simulink model "synRelSimuLutObs"  (R2023b)
settings: Solver=ode4  StartTime=0.0  StopTime=scenario.stopTime  FixedStep=Ts  RelTol=1e-4
values from neighbouring files (symbols this model uses):
  motor = setMotorParameters("SynRelLaplace")    [initSimulinkObs.m]    (also in setMotorParameters.m = struct)
  scenario = struct    [initSimulinkObs.m]
  trajectory = lutData.trajectory    [initSimulinkObs.m]    (also in test_cartos.m = load('synRelSimuLutData.mat').trajectory)
  Ts = 1e-4    (= 0.0001)    [initSimulinkObs.m]
undefined symbols (not defined in the file or in its folder): control, DiscIntNeverNeededParam, inverter, math, observer
libraries: simulink x2, slpidlib x1
settings Model: Creator=promu  LastModifiedBy=peralezADM
settings OptimizationCC: ReuseModelBlockBuffer=off
settings ModelReferenceCC: EnableRefExpFcnMdlSchedulingChecks=on

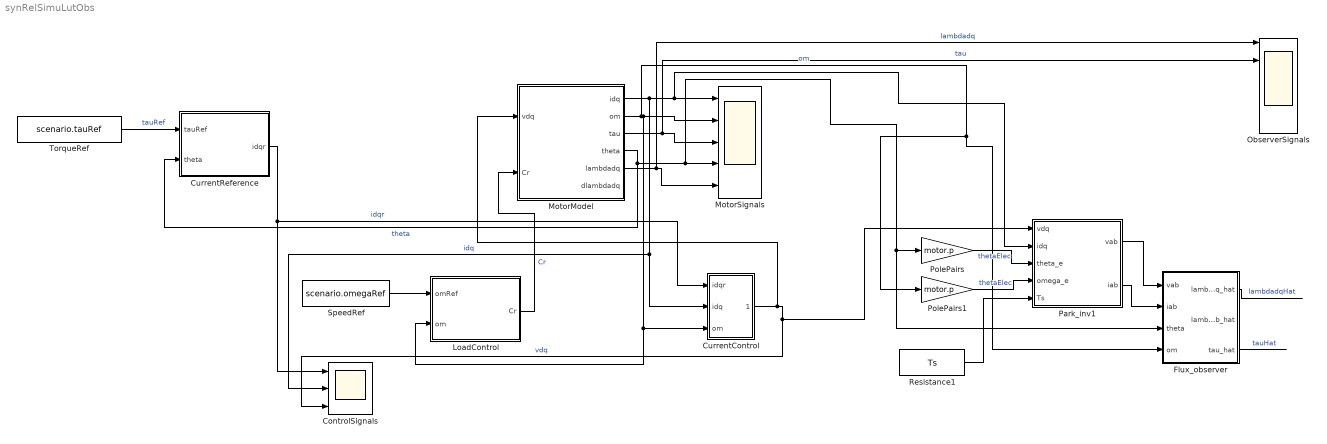
== system synRelSimuLutObs ==
  ControlSignals : Scope  NumInputPorts=3
  CurrentControl : Subsystem
  CurrentReference : Subsystem
  Flux_observer : Subsystem
  LoadControl : Subsystem
  MotorModel : Subsystem
  MotorSignals : Scope  NumInputPorts=5
  ObserverSignals : Scope  NumInputPorts=11
  Park_inv1 : MATLAB Function  TreatAsAtomicUnit=on
  PolePairs : Gain  Gain=motor.p
  PolePairs1 : Gain  Gain=motor.p
  Resistance1 : Constant  Value=Ts
  SpeedRef : Constant  Value=scenario.omegaRef
  TorqueRef : Constant  Value=scenario.tauRef
  wires:
  TorqueRef/1 -> CurrentReference/1(tauRef)  "tauRef"
  LoadControl/1(Cr) -> MotorModel/2(Cr)  "Cr"
  CurrentReference/1(idqr) -> CurrentControl/1(idqr), ControlSignals/1  "idqr"
  CurrentControl/1(v_dq) -> Park_inv1/1(vdq), ControlSignals/3, MotorModel/1(vdq)  "vdq"
  MotorModel/4(theta) -> CurrentReference/2(theta), MotorSignals/4, Flux_observer/3(theta), PolePairs/1  "theta"
  MotorModel/5(lambdadq) -> MotorSignals/5, ObserverSignals/1  "lambdadq"
  MotorModel/3(tau) -> ObserverSignals/3, MotorSignals/3  "tau"
  MotorModel/2(om) -> LoadControl/2(om), CurrentControl/3(om), MotorSignals/2, PolePairs1/1, Flux_observer/4(om)  "om"
  MotorModel/1(idq) -> ControlSignals/2, CurrentControl/2(idq), MotorSignals/1, Park_inv1/2(idq)  "idq"
  SpeedRef/1 -> LoadControl/1(omRef)
  Park_inv1/1(vab) -> Flux_observer/1(vab)
  PolePairs/1 -> Park_inv1/3(theta_e)  "thetaElec"
  Flux_observer/1(lambda_dq_hat) -> ?  "lambdadqHat"
  PolePairs1/1 -> Park_inv1/4(omega_e)  "thetaElec"
  Resistance1/1 -> Park_inv1/5(Ts)
  Park_inv1/2(iab) -> Flux_observer/2(iab)
  Flux_observer/3(tau_hat) -> ?  "tauHat"

== system synRelSimuLutObs/CurrentControl ==
  idqr : Inport
  idq : Inport  Port=2
  om : Inport  Port=3
  FeedbackLinearization : Subsystem
  GainElec : Constant  Value=control.kElecd  OutDataTypeStr=double
  PiCurrentLoops : Subsystem
      settings: PortSchema="{\"entries\":[{\"content\":{\"sides\":[{\"content\":{\"connectorIds\":[\"In1\",\"In2\",\"In3\"]},\"type\":\"ConnectorPlacement.EquallySpacedRectSide\",\"uuid\":\"0dd1bd5c-4f2d-4a51-9bc2-8bf74640d4ff\"},{\"content\":{\"connectorIds\":[\"Out1\"],\"side\":\"RIGHT\"},\"type\":\"ConnectorPlacement.EquallySpacedRectSide\",\"uuid\":\"9ff54608-efe8-47a2-97c0-1c2807ae0451\"},{\"content\":{\"connectorIds\":[],\"side\":\"TOP\"},\"type\":\"ConnectorPlacement.EquallySpacedRectSide\",\"uuid\":\"a5b0a1bc-2629-443b-a6ad-4c332df72e2c\"},{\"content\":{\"connectorIds\":[\"In4\",\"In5\"],\"side\":\"BOTTOM\"},\"type\":\"ConnectorPlacement.EquallySpacedRectSide\",\"uuid\":\"e8d63822-9705-4716-821c-9412f2966827\"},{\"content\":{\"connectorIds\":[],\"side\":\"HIDDEN\"},\"type\":\"ConnectorPlacement.EquallySpacedRectSide\",\"uuid\":\"63401b5c-75e9-49e9-aa08-12658d9987d3\"}]},\"type\":\"ConnectorPlacement.EquallySpacedConnector\",\"uuid\":\"d3f45542-3ea7-483a-a2ee-6c72d9ae8820\"}],\"packageUris\":[\"http://schema.mathworks.com/mf0/Connector/R2020b\"],\"version\":\"1.0\"}"
  VoltageSaturation : Subsystem
  v_dq : Outport
  wires:
  VoltageSaturation/1(vdqsat) -> v_dq/1
  FeedbackLinearization/1(v_dq) -> VoltageSaturation/1(vdq)
  idq/1 -> FeedbackLinearization/1(idq), PiCurrentLoops/2(idq)
  PiCurrentLoops/1(v_dq) -> FeedbackLinearization/2(udq)
  idqr/1 -> PiCurrentLoops/1(idqr)
  om/1 -> FeedbackLinearization/3(om)
  GainElec/1 -> PiCurrentLoops/5(Keq), PiCurrentLoops/4(Ked)
  VoltageSaturation/2(saturation) -> PiCurrentLoops/3(saturation)

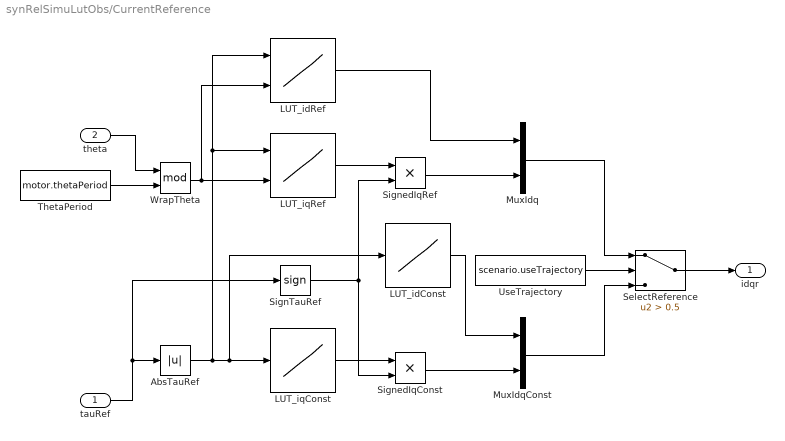
== system synRelSimuLutObs/CurrentReference ==
  tauRef : Inport
  theta : Inport  Port=2
  AbsTauRef : Abs  SaturateOnIntegerOverflow=off
  LUT_idConst : Lookup_n-D  NumberOfTableDimensions=1  BreakpointsForDimension1=trajectory.tauRef  Table=trajectory.idConst  ExtrapMethod=Clip  InternalRulePriority=Speed  RndMeth=Simplest
  LUT_idRef : Lookup_n-D  BreakpointsForDimension1=trajectory.tauRef  BreakpointsForDimension2=trajectory.theta  Table=trajectory.id  ExtrapMethod=Clip  InternalRulePriority=Speed  RndMeth=Simplest
      settings: InputPortMap=u0,u1
  LUT_iqConst : Lookup_n-D  NumberOfTableDimensions=1  BreakpointsForDimension1=trajectory.tauRef  Table=trajectory.iqConst  ExtrapMethod=Clip  InternalRulePriority=Speed  RndMeth=Simplest
  LUT_iqRef : Lookup_n-D  BreakpointsForDimension1=trajectory.tauRef  BreakpointsForDimension2=trajectory.theta  Table=trajectory.iq  ExtrapMethod=Clip  InternalRulePriority=Speed  RndMeth=Simplest
      settings: InputPortMap=u0,u1
  MuxIdq : Mux  Inputs=2
  MuxIdqConst : Mux  Inputs=2
  SelectReference : Switch  Criteria=u2 > Threshold  Threshold=0.5  SaturateOnIntegerOverflow=off  InputSameDT=off
  SignTauRef : Signum
  SignedIqConst : Product
  SignedIqRef : Product
  ThetaPeriod : Constant  Value=motor.thetaPeriod
  UseTrajectory : Constant  Value=scenario.useTrajectory
  WrapTheta : Math  Operator=mod
  idqr : Outport
  wires:
  MuxIdqConst/1 -> SelectReference/3
  UseTrajectory/1 -> SelectReference/2
  theta/1 -> WrapTheta/1
  SelectReference/1 -> idqr/1
  LUT_idConst/1 -> MuxIdqConst/1
  ThetaPeriod/1 -> WrapTheta/2
  tauRef/1 -> AbsTauRef/1, SignTauRef/1
  LUT_idRef/1 -> MuxIdq/1
  SignedIqConst/1 -> MuxIdqConst/2
  WrapTheta/1 -> LUT_iqRef/2, LUT_idRef/2
  AbsTauRef/1 -> LUT_iqConst/1, LUT_idConst/1, LUT_idRef/1, LUT_iqRef/1
  LUT_iqRef/1 -> SignedIqRef/1
  LUT_iqConst/1 -> SignedIqConst/1
  SignedIqRef/1 -> MuxIdq/2
  SignTauRef/1 -> SignedIqRef/2, SignedIqConst/2
  MuxIdq/1 -> SelectReference/1

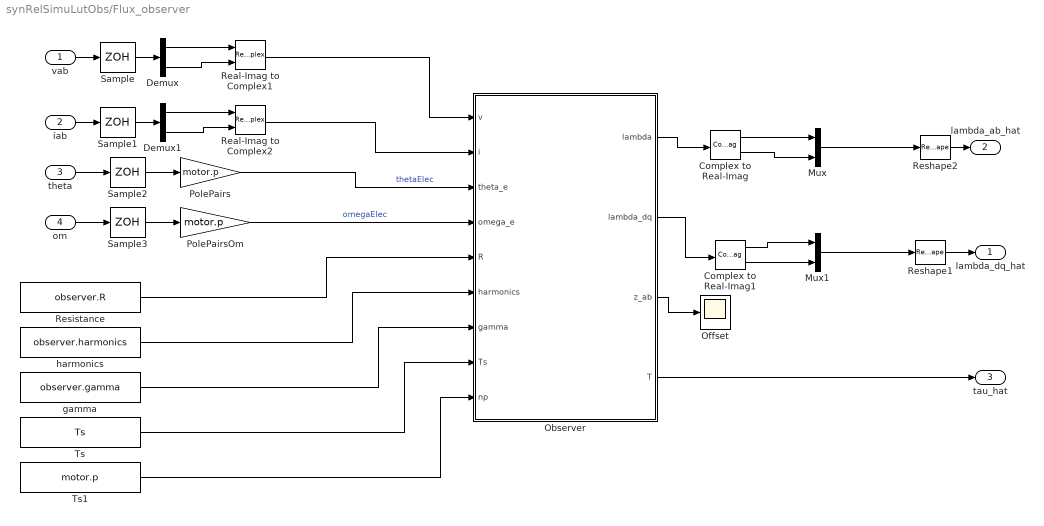
== system synRelSimuLutObs/Flux_observer ==
  vab : Inport
  iab : Inport  Port=2
  theta : Inport  Port=3
  om : Inport  Port=4
  Complex to Real-Imag : ComplexToRealImag
  Complex to Real-Imag1 : ComplexToRealImag
  Demux : Demux  Outputs=2
  Demux1 : Demux  Outputs=2
  Mux : Mux  Inputs=2
  Mux1 : Mux  Inputs=2
  Observer : MATLAB Function  TreatAsAtomicUnit=on
  Offset : Scope
  PolePairs : Gain  Gain=motor.p
  PolePairsOm : Gain  Gain=motor.p
  Real-Imag to Complex1 : RealImagToComplex
  Real-Imag to Complex2 : RealImagToComplex
  Reshape1 : Reshape
  Reshape2 : Reshape
  Resistance : Constant  Value=observer.R
  Sample{,1..3} (4 alike) : ZeroOrderHold  SampleTime=Ts
  Ts : Constant  Value=Ts
  Ts1 : Constant  Value=motor.p
  gamma : Constant  Value=observer.gamma
  harmonics : Constant  Value=observer.harmonics
  lambda_dq_hat : Outport
  lambda_ab_hat : Outport  Port=2
  tau_hat : Outport  Port=3
  wires:
  theta/1 -> Sample2/1
  om/1 -> Sample3/1
  PolePairsOm/1 -> Observer/4(omega_e)  "omegaElec"
  Resistance/1 -> Observer/5(R)
  harmonics/1 -> Observer/6(harmonics)
  gamma/1 -> Observer/7(gamma)
  PolePairs/1 -> Observer/3(theta_e)  "thetaElec"
  Mux1/1 -> Reshape1/1
  Reshape1/1 -> lambda_dq_hat/1
  Reshape2/1 -> lambda_ab_hat/1
  vab/1 -> Sample/1
  Demux/2 -> Real-Imag to Complex1/2
  Demux/1 -> Real-Imag to Complex1/1
  Real-Imag to Complex1/1 -> Observer/1(v)
  iab/1 -> Sample1/1
  Demux1/1 -> Real-Imag to Complex2/1
  Demux1/2 -> Real-Imag to Complex2/2
  Real-Imag to Complex2/1 -> Observer/2(i)
  Observer/1(lambda) -> Complex to Real-Imag/1
  Complex to Real-Imag/2 -> Mux/2
  Complex to Real-Imag/1 -> Mux/1
  Ts/1 -> Observer/8(Ts)
  Mux/1 -> Reshape2/1
  Observer/2(lambda_dq) -> Complex to Real-Imag1/1
  Complex to Real-Imag1/2 -> Mux1/2
  Complex to Real-Imag1/1 -> Mux1/1
  Observer/3(z_ab) -> Offset/1
  Sample/1 -> Demux/1
  Sample1/1 -> Demux1/1
  Sample2/1 -> PolePairs/1
  Sample3/1 -> PolePairsOm/1
  Ts1/1 -> Observer/9(np)
  Observer/4(T) -> tau_hat/1

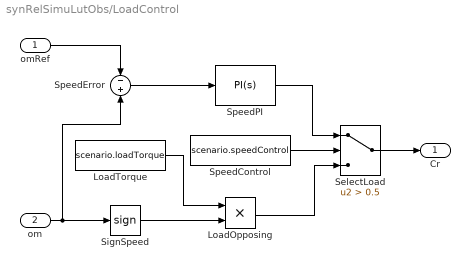
== system synRelSimuLutObs/LoadControl ==
  omRef : Inport
  om : Inport  Port=2
  LoadOpposing : Product
  LoadTorque : Constant  Value=scenario.loadTorque
  SelectLoad : Switch  Criteria=u2 > Threshold  Threshold=0.5  SaturateOnIntegerOverflow=off  InputSameDT=off
  SignSpeed : Signum
  SpeedControl : Constant  Value=scenario.speedControl
  SpeedError : Sum  Inputs=-+
  SpeedPI : slpidlib/PID Controller  Controller=PI  Form=Parallel  TimeDomain=Continuous-time  UseExternalTs=off  SampleTime=-1  IntegratorMethod=Forward Euler  FilterMethod=Forward Euler  ControllerParametersSource=internal  P=control.kpSpeed  I=control.kiSpeed  UseKiTs=off  D=0  N=100  UseFilter=on  TunerSelectOption=Transfer Function Based (PID Tuner App)  InitialConditionSource=internal  InitialConditionForIntegrator=0  InitialConditionForFilter=0  DifferentiatorICPrevScaledInput=0  ExternalReset=none  TrackingMode=off  Kt=1  LimitOutput=on  SatLimitsSource=internal  UpperSaturationLimit=scenario.loadMax  LowerSaturationLimit=-scenario.loadMax  LinearizeAsGain=on  AntiWindupMode=clamping  Kb=1  LimitIntegrator=off  UpperIntegratorSaturationLimit=inf  LowerIntegratorSaturationLimit=-inf  POutMin=[]  POutMax=[]  IOutMin=[]  IOutMax=[]  DOutMin=[]  DOutMax=[]  NOutMin=[]  NOutMax=[]  SumOutMin=[]  SumOutMax=[]  SaturationOutMin=[]  SaturationOutMax=[]  PParamMin=[]  PParamMax=[]  IParamMin=[]  IParamMax=[]  DParamMin=[]  DParamMax=[]  NParamMin=[]  NParamMax=[]  KbParamMin=[]  KbParamMax=[]  KtParamMin=[]  KtParamMax=[]  KbOutMin=[]  KbOutMax=[]  KtOutMin=[]  KtOutMax=[]  IntegratorOutMin=[]  IntegratorOutMax=[]  FilterOutMin=[]  FilterOutMax=[]  SumI1OutMin=[]  SumI1OutMax=[]  SumI2OutMin=[]  SumI2OutMax=[]  SumI3OutMin=[]  SumI3OutMax=[]  SumI4OutMin=[]  SumI4OutMax=[]  SumDOutMin=[]  SumDOutMax=[]  DifferentiatorOutMin=[]  DifferentiatorOutMax=[]  FilterDiffOutCoefMin=[]  FilterDiffOutCoefMax=[]  ReciprocalOutMin=[]  ReciprocalOutMax=[]  SumDenOutMin=[]  SumDenOutMax=[]  SumNumOutMin=[]  SumNumOutMax=[]  DivideOutMin=[]  DivideOutMax=[]  UdiffTsProdOutMin=[]  UdiffTsProdOutMax=[]  NTsProdOutMin=[]  NTsProdOutMax=[]  UintegralTsProdOutMin=[]  UintegralTsProdOutMax=[]  UngainTsProdOutMin=[]  UngainTsProdOutMax=[]  ClampingZeroOutDataTypeStr=Inherit: Inherit via back propagation  ClampingZeroOutMin=[]  ClampingZeroOutMax=[]  FilterDenConstantOutDataTypeStr=Inherit: Inherit via back propagation  FilterDenConstantOutMin=[]  FilterDenConstantOutMax=[]  PCopyOutDataTypeStr=Inherit: Inherit via back propagation  PCopyOutMin=[]  PCopyOutMax=[]  NCopyOutDataTypeStr=Inherit: Inherit via back propagation  NCopyOutMin=[]  NCopyOutMax=[]  IntegratorContinuousStateAttributes=''  IntegratorStateMustResolveToSignalObject=off  IntegratorRTWStateStorageClass=Auto  FilterContinuousStateAttributes=''  FilterStateMustResolveToSignalObject=off  FilterRTWStateStorageClass=Auto  ParallelPVariant=InternalParameters  IdealPVariant=Disabled  IVariant=InternalParameters  DVariant=Disabled  IntegratorVariant=Continuous  SatVariant=Enabled  AWVariant=ContClampingParallel  PCopyVariant=Disabled  TRVariant=Disabled  FdbkBlocksVariant=Forward  IdealPFdbkVariant=Disabled  SatFdbkVariant=Disabled  DerivativeFilterVariant=Disabled  NVariant=Disabled  NCopyVariant=Disabled_SignalSpec  FilterICVariant=Disabled  IntegratorICVariant=InternalICs  ExternalResetVariant=Disabled  TRSumVariant=Passthrough  SumFdbkVariant=Disabled  SumVariant=Sum_PI  TsampFilterVariant=InternalTs  TsampNgainVariant=Passthrough  TsampIntegralVariant=Disabled_SignalSpec  ExternalSaturationOutDataTypeStr=Inherit: Same as second input
  Cr : Outport
  wires:
  SelectLoad/1 -> Cr/1
  SpeedPI/1 -> SelectLoad/1
  SignSpeed/1 -> LoadOpposing/2
  LoadOpposing/1 -> SelectLoad/3
  LoadTorque/1 -> LoadOpposing/1
  SpeedError/1 -> SpeedPI/1
  om/1 -> SignSpeed/1, SpeedError/2
  SpeedControl/1 -> SelectLoad/2
  omRef/1 -> SpeedError/1

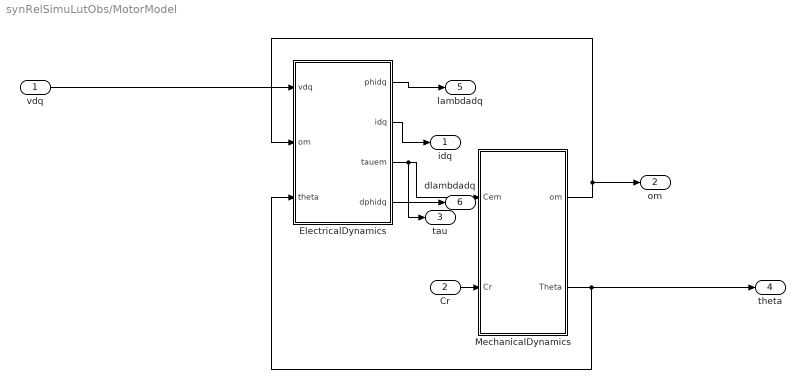
== system synRelSimuLutObs/MotorModel ==
  vdq : Inport
  Cr : Inport  Port=2
  ElectricalDynamics : Subsystem
  MechanicalDynamics : Subsystem
  idq : Outport
  om : Outport  Port=2
  tau : Outport  Port=3
  theta : Outport  Port=4
  lambdadq : Outport  Port=5
  dlambdadq : Outport  Port=6
  wires:
  vdq/1 -> ElectricalDynamics/1(vdq)
  ElectricalDynamics/2(idq) -> idq/1
  Cr/1 -> MechanicalDynamics/2(Cr)
  ElectricalDynamics/3(tauem) -> MechanicalDynamics/1(Cem), tau/1
  MechanicalDynamics/1(om) -> ElectricalDynamics/2(om), om/1
  MechanicalDynamics/2(Theta) -> ElectricalDynamics/3(theta), theta/1
  ElectricalDynamics/1(phidq) -> lambdadq/1
  ElectricalDynamics/4(dphidq) -> dlambdadq/1

== system synRelSimuLutObs/CurrentControl/FeedbackLinearization ==
  idq : Inport
  udq : Inport  Port=2
  om : Inport  Port=3
  Add : Sum
  Gain : Gain  Gain=math.J*motor.Ldq  Multiplication=Matrix(K*u)
  Gain1 : Gain  Gain=motor.p
  Product : Product
  v_dq : Outport  VectorParamsAs1DForOutWhenUnconnected=off
  wires:
  idq/1 -> Gain/1
  Gain/1 -> Product/1
  Add/1 -> v_dq/1
  udq/1 -> Add/1
  om/1 -> Gain1/1
  Gain1/1 -> Product/2
  Product/1 -> Add/2

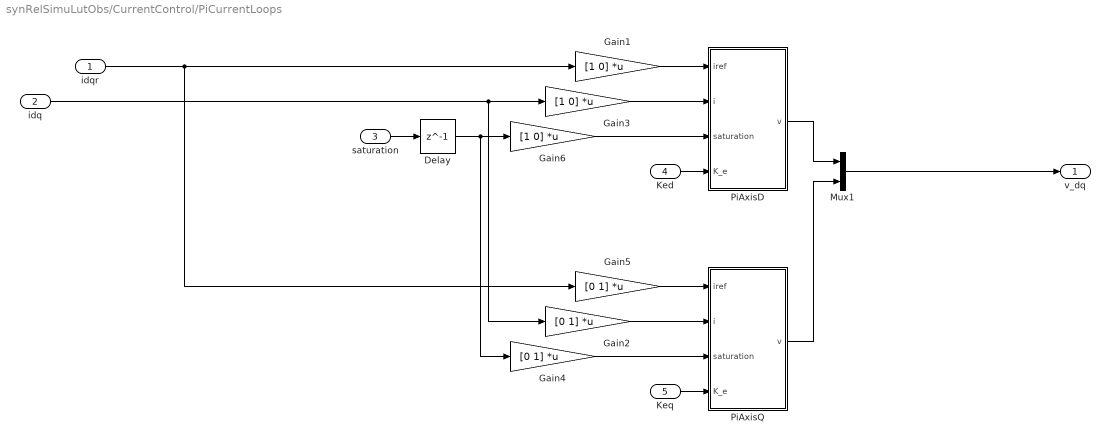
== system synRelSimuLutObs/CurrentControl/PiCurrentLoops ==
  idqr : Inport
  idq : Inport  Port=2
  saturation : Inport  Port=3
  Ked : Inport  Port=4
  Keq : Inport  Port=5
  Delay : Delay  DelayLength=1
  Gain1 : Gain  Gain=[1 0]  Multiplication=Matrix(K*u)  OutDataTypeStr=Inherit: Same as input
  Gain2 : Gain  Gain=[0 1]  Multiplication=Matrix(K*u)  OutDataTypeStr=Inherit: Same as input
  Gain3 : Gain  Gain=[1 0]  Multiplication=Matrix(K*u)  OutDataTypeStr=Inherit: Same as input
  Gain4 : Gain  Gain=[0 1]  Multiplication=Matrix(K*u)  OutDataTypeStr=Inherit: Same as input
  Gain5 : Gain  Gain=[0 1]  Multiplication=Matrix(K*u)  OutDataTypeStr=Inherit: Same as input
  Gain6 : Gain  Gain=[1 0]  Multiplication=Matrix(K*u)  OutDataTypeStr=Inherit: Same as input
  Mux1 : Mux  Inputs=2
  PiAxisD : Subsystem
  PiAxisQ : Subsystem
  v_dq : Outport  VectorParamsAs1DForOutWhenUnconnected=off
  wires:
  Gain4/1 -> PiAxisQ/3(saturation)
  Gain6/1 -> PiAxisD/3(saturation)
  Delay/1 -> Gain6/1, Gain4/1
  Mux1/1 -> v_dq/1
  Gain2/1 -> PiAxisQ/2(i)
  Gain3/1 -> PiAxisD/2(i)
  idq/1 -> Gain3/1, Gain2/1
  PiAxisD/1(v) -> Mux1/1
  PiAxisQ/1(v) -> Mux1/2
  saturation/1 -> Delay/1
  idqr/1 -> Gain5/1, Gain1/1
  Gain5/1 -> PiAxisQ/1(iref)
  Gain1/1 -> PiAxisD/1(iref)
  Ked/1 -> PiAxisD/4(K_e)
  Keq/1 -> PiAxisQ/4(K_e)

== system synRelSimuLutObs/CurrentControl/VoltageSaturation ==
  vdq : Inport
  Divide : Product  Inputs=*/
  Gain : Gain  Gain=inverter.vMax
  Norm L2 : Subsystem
  Sum : Sum  Inputs=|+-
  Switch : Switch  Criteria=u2 > Threshold  Threshold=inverter.vMax  SaturateOnIntegerOverflow=off  InputSameDT=off
  vdqsat : Outport  VectorParamsAs1DForOutWhenUnconnected=off
  saturation : Outport  Port=2  VectorParamsAs1DForOutWhenUnconnected=off
  wires:
  Gain/1 -> Switch/1
  Norm L2/1(y) -> Divide/2, Switch/2
  Divide/1 -> Gain/1
  Switch/1 -> Sum/2, vdqsat/1
  vdq/1 -> Norm L2/1(In1), Divide/1, Sum/1, Switch/3
  Sum/1 -> saturation/1

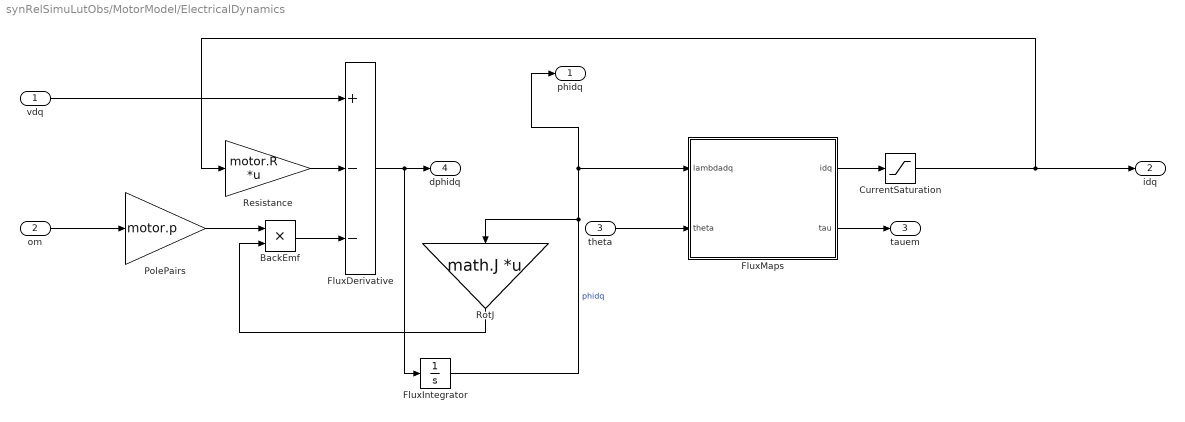
== system synRelSimuLutObs/MotorModel/ElectricalDynamics ==
  vdq : Inport
  om : Inport  Port=2
  theta : Inport  Port=3
  BackEmf : Product
  CurrentSaturation : Saturate  UpperLimit=motor.lutInv.iMax  LowerLimit=-motor.lutInv.iMax
  FluxDerivative : Sum  Inputs=+--
  FluxIntegrator : Integrator  InitialCondition=[0 0]  LimitOutput=on  UpperSaturationLimit=[max(motor.lutInv.lambdad) max(motor.lutInv.lambdaq)]  LowerSaturationLimit=-[max(motor.lutInv.lambdad) max(motor.lutInv.lambdaq)]
  FluxMaps : Subsystem
  PolePairs : Gain  Gain=motor.p
  Resistance : Gain  Gain=motor.R  Multiplication=Matrix(K*u)
  RotJ : Gain  Gain=math.J  Multiplication=Matrix(K*u)
  phidq : Outport
  idq : Outport  Port=2
  tauem : Outport  Port=3
  dphidq : Outport  Port=4
  wires:
  RotJ/1 -> BackEmf/2
  om/1 -> PolePairs/1
  PolePairs/1 -> BackEmf/1
  BackEmf/1 -> FluxDerivative/3
  vdq/1 -> FluxDerivative/1
  Resistance/1 -> FluxDerivative/2
  FluxMaps/1(idq) -> CurrentSaturation/1
  CurrentSaturation/1 -> Resistance/1, idq/1
  theta/1 -> FluxMaps/2(theta)
  FluxMaps/2(tau) -> tauem/1
  FluxDerivative/1 -> dphidq/1, FluxIntegrator/1
  FluxIntegrator/1 -> FluxMaps/1(lambdadq), phidq/1, RotJ/1  "phidq"

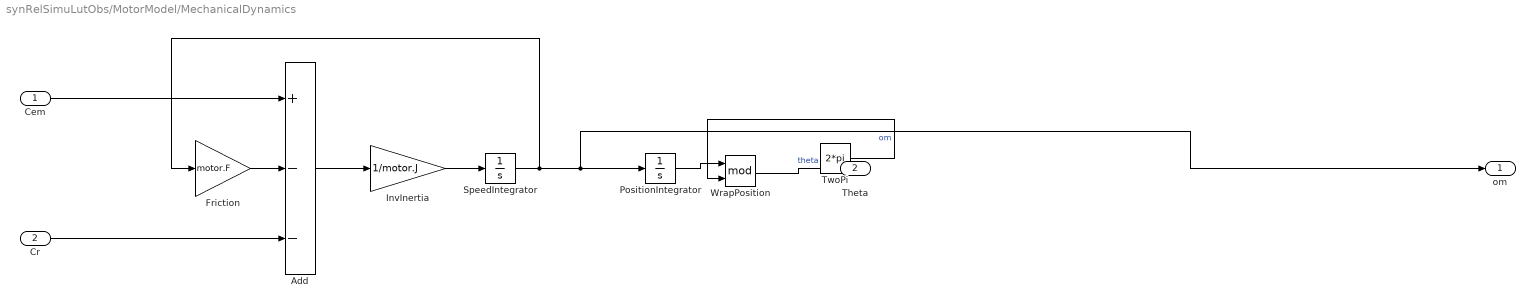
== system synRelSimuLutObs/MotorModel/MechanicalDynamics ==
  Cem : Inport
  Cr : Inport  Port=2
  Add : Sum  Inputs=+--
  Friction : Gain  Gain=motor.F
  InvInertia : Gain  Gain=1/motor.J
  PositionIntegrator : Integrator  InitialCondition=scenario.theta0
  SpeedIntegrator : Integrator  InitialCondition=scenario.omega0
  TwoPi : Constant  Value=2*pi
  WrapPosition : Math  Operator=mod
  om : Outport
  Theta : Outport  Port=2  VectorParamsAs1DForOutWhenUnconnected=off
  wires:
  InvInertia/1 -> SpeedIntegrator/1
  Friction/1 -> Add/2
  Cem/1 -> Add/1
  Cr/1 -> Add/3
  Add/1 -> InvInertia/1
  WrapPosition/1 -> Theta/1  "theta"
  TwoPi/1 -> WrapPosition/2
  PositionIntegrator/1 -> WrapPosition/1
  SpeedIntegrator/1 -> om/1, PositionIntegrator/1, Friction/1  "om"

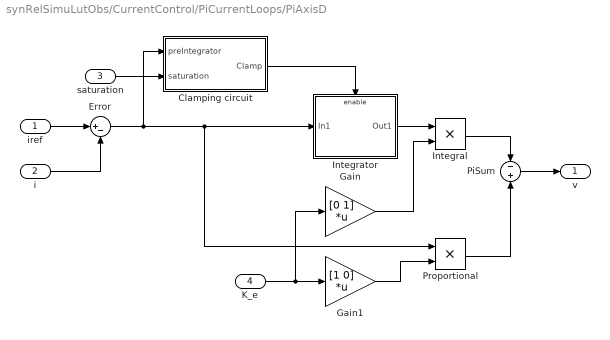
== system synRelSimuLutObs/CurrentControl/PiCurrentLoops/PiAxisD ==
  iref : Inport
  i : Inport  Port=2
  saturation : Inport  Port=3
  K_e : Inport  Port=4
  Clamping circuit : Subsystem
  Error : Sum  Inputs=|+-
  Gain : Gain  Gain=[0 1]  Multiplication=Matrix(K*u)
  Gain1 : Gain  Gain=[1 0]  Multiplication=Matrix(K*u)
  Integral : Product
  Integrator : Subsystem
  PiSum : Sum  Inputs=-+  OutDataTypeStr=double  SaturateOnIntegerOverflow=on
  Proportional : Product
  v : Outport  VectorParamsAs1DForOutWhenUnconnected=off
  wires:
  PiSum/1 -> v/1
  Integral/1 -> PiSum/1
  Proportional/1 -> PiSum/2
  Gain1/1 -> Proportional/2
  Gain/1 -> Integral/2
  Integrator/1(Out1) -> Integral/1
  K_e/1 -> Gain/1, Gain1/1
  saturation/1 -> Clamping circuit/2(saturation)
  Clamping circuit/1(Clamp) -> Integrator/Enable
  Error/1 -> Integrator/1(In1), Proportional/1, Clamping circuit/1(preIntegrator)
  i/1 -> Error/2
  iref/1 -> Error/1

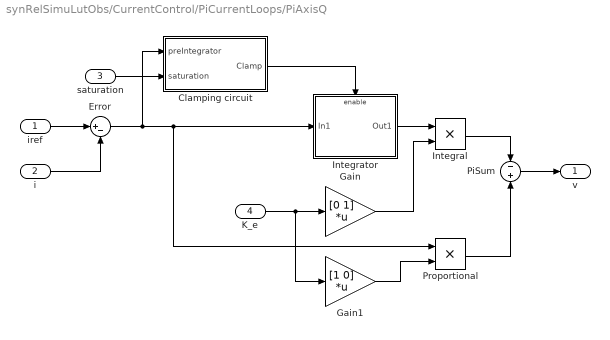
== system synRelSimuLutObs/CurrentControl/PiCurrentLoops/PiAxisQ ==
  iref : Inport
  i : Inport  Port=2
  saturation : Inport  Port=3
  K_e : Inport  Port=4
  Clamping circuit : Subsystem
  Error : Sum  Inputs=|+-
  Gain : Gain  Gain=[0 1]  Multiplication=Matrix(K*u)
  Gain1 : Gain  Gain=[1 0]  Multiplication=Matrix(K*u)
  Integral : Product
  Integrator : Subsystem
  PiSum : Sum  Inputs=-+  OutDataTypeStr=double  SaturateOnIntegerOverflow=on
  Proportional : Product
  v : Outport  VectorParamsAs1DForOutWhenUnconnected=off
  wires:
  Integral/1 -> PiSum/1
  Gain/1 -> Integral/2
  Gain1/1 -> Proportional/2
  K_e/1 -> Gain1/1, Gain/1
  Clamping circuit/1(Clamp) -> Integrator/Enable
  Error/1 -> Integrator/1(In1), Proportional/1, Clamping circuit/1(preIntegrator)
  saturation/1 -> Clamping circuit/2(saturation)
  PiSum/1 -> v/1
  i/1 -> Error/2
  Proportional/1 -> PiSum/2
  Integrator/1(Out1) -> Integral/1
  iref/1 -> Error/1

== system synRelSimuLutObs/CurrentControl/VoltageSaturation/Norm L2 ==
  In1 : Inport
  Dot Product : DotProduct  OutDataTypeStr=Inherit: Inherit via internal rule
  Sqrt : Sqrt
  y : Outport
  wires:
  Sqrt/1 -> y/1
  Dot Product/1 -> Sqrt/1
  In1/1 -> Dot Product/2, Dot Product/1

== system synRelSimuLutObs/MotorModel/ElectricalDynamics/FluxMaps ==
  lambdadq : Inport
  theta : Inport  Port=2
  InverseFluxMap : Subsystem
  TorqueMap : Subsystem
  idq : Outport
  tau : Outport  Port=2
  wires:
  TorqueMap/1(tau) -> tau/1
  InverseFluxMap/1(idq) -> idq/1, TorqueMap/1(idq)
  theta/1 -> InverseFluxMap/2(theta), TorqueMap/2(theta)
  lambdadq/1 -> InverseFluxMap/1(lambdadq)

== system synRelSimuLutObs/CurrentControl/PiCurrentLoops/PiAxisD/Clamping circuit ==
  note: The clamping enable or disable the integral action.
  preIntegrator : Inport  DisableCoverage=on
  saturation : Inport  DisableCoverage=on  Port=2
  Compare To Zero1 : simulink/Logic and Bit Operations/Compare To Zero  relop=<=  OutDataTypeStr=boolean
  Multiply : Product
  Clamp : Outport  DisableCoverage=on  VectorParamsAs1DForOutWhenUnconnected=off
  wires:
  preIntegrator/1 -> Multiply/2
  saturation/1 -> Multiply/1
  Multiply/1 -> Compare To Zero1/1
  Compare To Zero1/1 -> Clamp/1

== system synRelSimuLutObs/CurrentControl/PiCurrentLoops/PiAxisD/Integrator ==
  In1 : Inport
  Enable : EnablePort
  Discrete-Time Integrator : DiscreteIntegrator  SampleTime=Ts  OutDataTypeStr=double  ICPrevOutput=DiscIntNeverNeededParam  ICPrevScaledInput=DiscIntNeverNeededParam
  Out1 : Outport  VectorParamsAs1DForOutWhenUnconnected=off
  wires:
  In1/1 -> Discrete-Time Integrator/1
  Discrete-Time Integrator/1 -> Out1/1

== system synRelSimuLutObs/CurrentControl/PiCurrentLoops/PiAxisQ/Clamping circuit ==
  note: The clamping enable or disable the integral action.
  preIntegrator : Inport  DisableCoverage=on
  saturation : Inport  DisableCoverage=on  Port=2
  Compare To Zero1 : simulink/Logic and Bit Operations/Compare To Zero  relop=<=  OutDataTypeStr=boolean
  Multiply : Product
  Clamp : Outport  DisableCoverage=on  VectorParamsAs1DForOutWhenUnconnected=off
  wires:
  preIntegrator/1 -> Multiply/2
  saturation/1 -> Multiply/1
  Multiply/1 -> Compare To Zero1/1
  Compare To Zero1/1 -> Clamp/1

== system synRelSimuLutObs/CurrentControl/PiCurrentLoops/PiAxisQ/Integrator ==
  In1 : Inport
  Enable : EnablePort
  Discrete-Time Integrator : DiscreteIntegrator  SampleTime=Ts  OutDataTypeStr=double  ICPrevOutput=DiscIntNeverNeededParam  ICPrevScaledInput=DiscIntNeverNeededParam
  Out1 : Outport  VectorParamsAs1DForOutWhenUnconnected=off
  wires:
  Discrete-Time Integrator/1 -> Out1/1
  In1/1 -> Discrete-Time Integrator/1

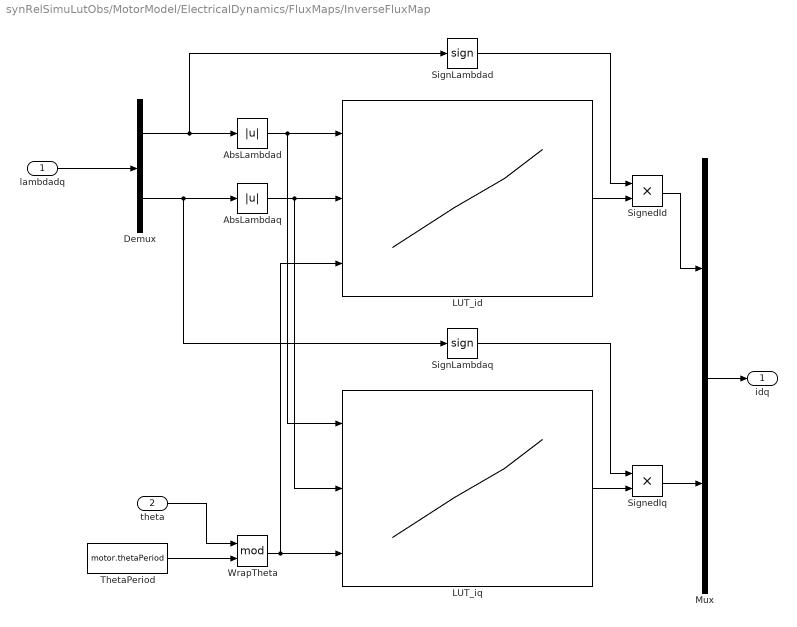
== system synRelSimuLutObs/MotorModel/ElectricalDynamics/FluxMaps/InverseFluxMap ==
  lambdadq : Inport
  theta : Inport  Port=2
  AbsLambdad : Abs  SaturateOnIntegerOverflow=off
  AbsLambdaq : Abs  SaturateOnIntegerOverflow=off
  Demux : Demux  Outputs=2
  LUT_id : Lookup_n-D  NumberOfTableDimensions=3  BreakpointsForDimension1=motor.lutInv.lambdad  BreakpointsForDimension2=motor.lutInv.lambdaq  BreakpointsForDimension3=motor.lutInv.theta  Table=motor.lutInv.id  InternalRulePriority=Speed  RndMeth=Simplest
      settings: InputPortMap=u0,u1,u2
  LUT_iq : Lookup_n-D  NumberOfTableDimensions=3  BreakpointsForDimension1=motor.lutInv.lambdad  BreakpointsForDimension2=motor.lutInv.lambdaq  BreakpointsForDimension3=motor.lutInv.theta  Table=motor.lutInv.iq  InternalRulePriority=Speed  RndMeth=Simplest
      settings: InputPortMap=u0,u1,u2
  Mux : Mux  Inputs=2
  SignLambdad : Signum
  SignLambdaq : Signum
  SignedId : Product
  SignedIq : Product
  ThetaPeriod : Constant  Value=motor.thetaPeriod
  WrapTheta : Math  Operator=mod
  idq : Outport
  wires:
  SignedIq/1 -> Mux/2
  lambdadq/1 -> Demux/1
  LUT_iq/1 -> SignedIq/2
  Demux/1 -> AbsLambdad/1, SignLambdad/1
  Demux/2 -> AbsLambdaq/1, SignLambdaq/1
  theta/1 -> WrapTheta/1
  LUT_id/1 -> SignedId/2
  Mux/1 -> idq/1
  ThetaPeriod/1 -> WrapTheta/2
  AbsLambdad/1 -> LUT_iq/1, LUT_id/1
  AbsLambdaq/1 -> LUT_iq/2, LUT_id/2
  SignLambdad/1 -> SignedId/1
  WrapTheta/1 -> LUT_iq/3, LUT_id/3
  SignedId/1 -> Mux/1
  SignLambdaq/1 -> SignedIq/1

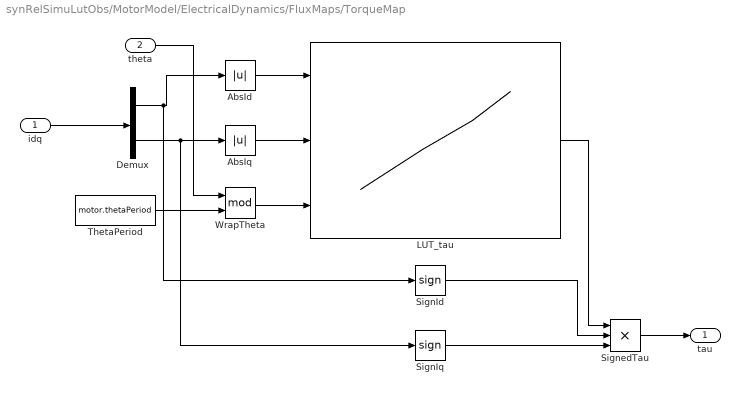
== system synRelSimuLutObs/MotorModel/ElectricalDynamics/FluxMaps/TorqueMap ==
  idq : Inport
  theta : Inport  Port=2
  AbsId : Abs  SaturateOnIntegerOverflow=off
  AbsIq : Abs  SaturateOnIntegerOverflow=off
  Demux : Demux  Outputs=2
  LUT_tau : Lookup_n-D  NumberOfTableDimensions=3  BreakpointsForDimension1=motor.lutTorque.id  BreakpointsForDimension2=motor.lutTorque.iq  BreakpointsForDimension3=motor.lutTorque.theta  Table=motor.lutTorque.tau  InternalRulePriority=Speed  RndMeth=Simplest
      settings: InputPortMap=u0,u1,u2
  SignId : Signum
  SignIq : Signum
  SignedTau : Product  Inputs=3
  ThetaPeriod : Constant  Value=motor.thetaPeriod
  WrapTheta : Math  Operator=mod
  tau : Outport
  wires:
  AbsIq/1 -> LUT_tau/2
  AbsId/1 -> LUT_tau/1
  ThetaPeriod/1 -> WrapTheta/2
  SignId/1 -> SignedTau/2
  Demux/2 -> AbsIq/1, SignIq/1
  SignedTau/1 -> tau/1
  Demux/1 -> AbsId/1, SignId/1
  SignIq/1 -> SignedTau/3
  theta/1 -> WrapTheta/1
  LUT_tau/1 -> SignedTau/1
  WrapTheta/1 -> LUT_tau/3
  idq/1 -> Demux/1

== matlab function synRelSimuLutObs/Flux_observer/Observer ==
  data: lambda output; v input; i input; theta_e input; omega_e input; R input; harmonics input; gamma input; Ts input; lambda_dq output; z_ab output; np input; T output
function [lambda, lambda_dq, z_ab, T] = flux_observer(v, i, theta_e, omega_e, R, harmonics, gamma, Ts, np)
	persistent p z i_dq_prev

    i_dq = i * exp(-1j * theta_e);

    if isempty(p)
        p = complex(zeros(1 + numel(harmonics), 1));
        z = 0 + 0j;
        i_dq_prev = i_dq;
        % Initial guess for [L_dd; L_qq; L_dq] in Henrys (e.g., [15mH; 8mH; -2mH])
        theta_L = [0.0367; 0.0163; 0.0];
    end
    
    h = harmonics(:); % Force harmonics regressor into a column vector
    phi = exp(1j * h * theta_e);
    lambda_0 = p(1);
    chi = p(2:end);

    %% 1. Faraday derivative & flux reconstruction
    z_dot = v - R * i;
    lambda = z + lambda_0;

    %% 2. Regressor and observation error
    z_est = -lambda_0 + sum(phi .* chi);
    err = z - z_est;

    %% 3. Adaptation dynamics
    kappa = omega_e * gamma;
    dot_lambda_0 = -kappa * err;
    dot_chi      =  kappa * conj(phi) * err;
    p_dot = [dot_lambda_0; dot_chi];

    p = p + Ts * p_dot;
    z = z + Ts * z_dot;

    lambda_dq = lambda * exp(-1j * theta_e);
    z_ab = z;

    %% 4. Torque computation
        
    % Angular derivative of lambda_dq
    % dlambda_dq_dtheta = sum(1j * (h - 1) .* phi .* chi) * exp(-1j * theta_e);
    dlambda_dq_dtheta = (z_dot / omega_e) * exp(-1j * theta_e) - 1j * lambda_dq;
     
    % Angular derivative of i_dq
    di_dq_dtheta = (i_dq - i_dq_prev) / (Ts * omega_e);
    i_dq_prev = i_dq;

    % Torque = Cross term + reluctance/harmonic term
    T_cross = imag(conj(lambda_dq) * i_dq);
    T_corr = 0.5 * real(conj(i_dq) * dlambda_dq_dtheta - conj(lambda_dq) * di_dq_dtheta);
    T = np * (T_cross + T_corr);
    
    
end

== matlab function synRelSimuLutObs/Park_inv1 ==
  data: vab output; vdq input; idq input; theta_e input; omega_e input; Ts input; iab output
function [vab, iab] = Park_inv(vdq, idq, theta_e, omega_e, Ts)
    theta_e_mid = mod(theta_e + 0.5 * Ts * omega_e, 2.0 * pi);

    vab = vdq;
	vab(1) = vdq(1) * cos(theta_e_mid) - vdq(2) * sin(theta_e_mid);
    vab(2) = vdq(1) * sin(theta_e_mid) + vdq(2) * cos(theta_e_mid);

    iab = idq;
	iab(1) = idq(1) * cos(theta_e_mid) - idq(2) * sin(theta_e_mid);
    iab(2) = idq(1) * sin(theta_e_mid) + idq(2) * cos(theta_e_mid);
end
